simulink model "BendingMoments"  (R2026a)
settings: Solver=ode4  StartTime=0  StopTime=30  FixedStep=0.005  RelTol=1e-6
undefined symbols (not defined in the file or in its folder): mp
libraries: simulink x4, aerolibasang x3, aerolibadyn x1, aerolibatmos2 x1
settings Model: Creator=slugg  LastModifiedBy=slugg
settings DataIOCC: ReturnWorkspaceOutputsName=tp2dc5d62c_f7e5_43a9_8206_2db448d4c4c5

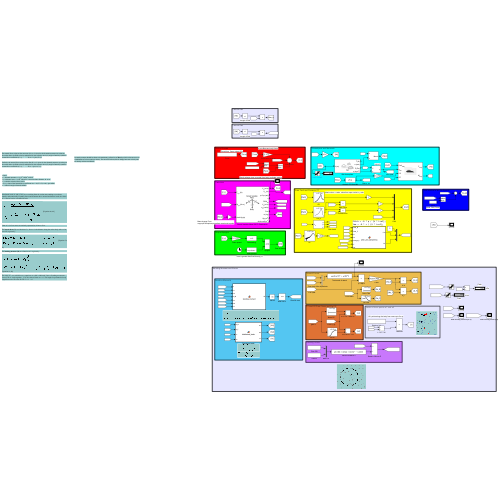
[thumbnail: Simulink's stored preview of the top-level diagram]
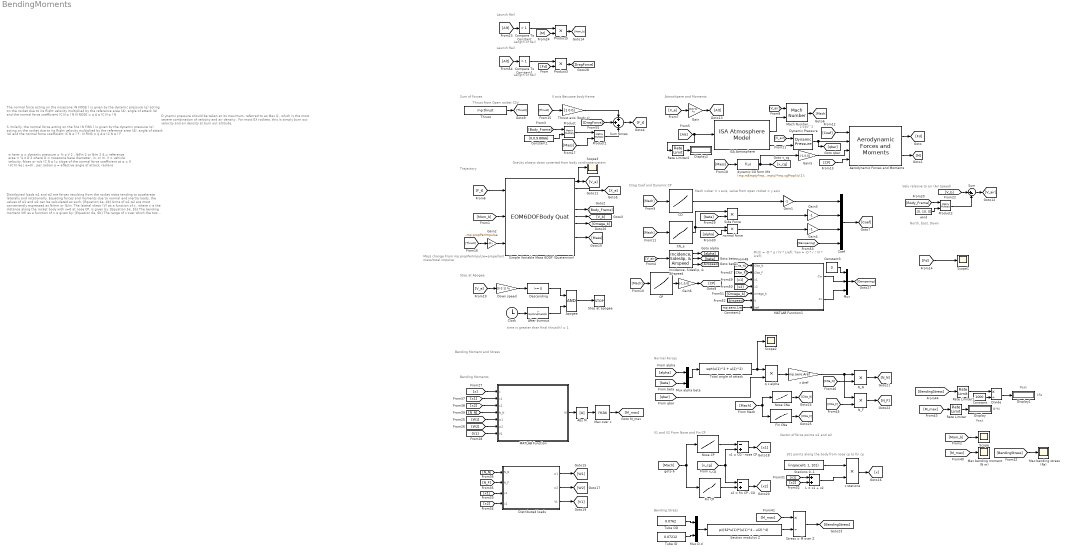
== system BendingMoments ==
  note: Bending Moment and Stress
  note: Pitch = -D * q / (V * Lref);
      | Yaw = -D * r / (V * Lref);
  note: Peak
  note: Peak
  note: N*M
  note: kPa
  note: Vector of force points w1 and w2
  note: 101 points along the body from nose cp to fin cp
  note: Normal Forces
  note: X1 and X2 From Nose and Fin CP
  note: Bending Moments
  note: Bending Stress
  note: Distributed loads w1 and w2 are forces resulting from the rocket mass tending to accelerate laterally and rotationally. Equating forces and moments due to normal and inertia loads, the values of w1 and w2 can be calculated as such:
      | [Equation 4a, 4b]
      | Units of w1,w2 are most conveniently expressed as N/mm or lb/in.
      | The lateral shear (V) as a function of x , where x is the distance along the rocket body with x=0 at nose CP, is given by:
      | [Equation 5a, 5b]
      | The bending moment (M) as a function of x is given by:
      | [Equation 6a, 6b]
      | The range of x over which the two equations are valid is indicated. Units of bending moment are N-mm or lb-in. In the equation , V1 is the value of shear at x=x1 . The length L represents the body length from nose CP to the fin CP: L = x1 + x2
  note: D ynamic pressure should be taken at its maximum, referred to as Max Q , which is the most severe combination of velocity and air density . For most EX rockets, this is simply burn out velocity and air density at burn out altitude.
  note: w here:
      | q = dynamic pressure = ½ ρ V 2 , lbf/in 2 or N/m 2
      | A = reference area = ¼ π D 2 where D = nosecone base diameter, in. or m.
      | V = vehicle velocity, ft/sec or m/s
      | (C N α )= slope of the normal force coefficient at α = 0 (∂C N /∂α | α=0) , per radian
      | α = effective angle of attack, radians
  note: S imilarly, the normal force acting on the fins (N FINS ) is given by the dynamic pressure (q) acting on the rocket due to its flight velocity multiplied by the reference area (A), angle of attack (α) and the normal force coefficient (C N α ) F : N FINS = q A α (C N α ) F
  note: The normal force acting on the nosecone (N NOSE ) is given by the dynamic pressure (q) acting on the rocket due to its flight velocity multiplied by the reference area (A), angle of attack (α) and the normal force coefficient (C N α ) N N NOSE = q A α (C N α ) N
  note: Mach nuber = x axis, value from open rocket = y axis
  note: time is greater than final thrust(t) = 1
  note: Mass change From
      | mp.propPerImpulse=propellant mass/total impulse
  note: X axis Becuase body frame
  note: Thrust from Open rocket CSV
  note: Gravity always down coverted from body cordinate system
  note: Length of Rail
  note: Launch Rail
  note: Velo relative to air (Air Speed)
  note: North, East, Down
  note: Atmoshpere and Moments
  note: Stop at Apogee
  note: Drag Coef and Dynamic CP
  note: Trajectory
  note: Sum of Forces
  note: 1/2pV^2
  note: Launch Rail
  note: Length of Rail
  Abs M : Abs  ZeroCross=off  SaturateOnIntegerOverflow=off
  "Aerodynamic Forces and Moments " : aerolibadyn/Aerodynamic Forces and Moments   inputAxes=Body  outputForceAxes=Body  outputMomentAxes=Body  S=mp.aero.Aref  b=mp.aero.Lref  cbar=mp.aero.Lref
  After burnout : simulink/Logic and Bit Operations/Compare To Constant  relop=>  const=mp.thrust(end,1)  OutDataTypeStr=boolean
  Apogee : Logic  AllPortsSameDT=off  OutDataTypeStr=boolean
  CD : Lookup_n-D  NumberOfTableDimensions=1  BreakpointsForDimension1=mp.aero.mach  Table=mp.aero.cd  ExtrapMethod=Clip  InternalRulePriority=Speed  RndMeth=Simplest
  CN_a : Lookup_n-D  NumberOfTableDimensions=1  BreakpointsForDimension1=[0.3, 0.4, 0.5, 0.6, 0.7, 0.8, 0.9, 1.0, 1.1, 1.2, 1.3, 1.4, 1.5, 1.6, 1.7]  Table=[9.822, 9.869, 9.931, 10.01, 10.108, 10.228, 10.374, 10.57, 10.867, 11.225, 11.509, 11.505, 10.944, 10.086, 9.424]  ExtrapMethod=Clip  InternalRulePriority=Speed  RndMeth=Simplest
  CP : Lookup_n-D  NumberOfTableDimensions=1  BreakpointsForDimension1=mp.aero.mach  Table=mp.aero.cp  ExtrapMethod=Clip  InternalRulePriority=Speed  RndMeth=Simplest
  Clock : Clock
  Coef : Mux  Inputs=[1,1,1,3]
  Compare To Constant : simulink/Logic and Bit Operations/Compare To Constant  relop=>  const=1  OutDataTypeStr=boolean
  Compare To Constant1 : simulink/Logic and Bit Operations/Compare To Constant  relop=>  const=1  OutDataTypeStr=boolean
  Constant : Constant  Value=1000
  Constant1 : Constant  Value=[0,0,9.8066]
  Constant2 : Constant  Value=mp.aero.Lref
  Constant3 : Constant  Value=0
  Descending : simulink/Logic and Bit Operations/Compare To Zero  relop=>=  OutDataTypeStr=boolean
  Display : Display
  Display1 : Display
  Display2 : Display
  Distributed loads : MATLAB Function  TreatAsAtomicUnit=on
  Divide : Product  Inputs=*/
  Down speed : Gain  Gain=[0 0 1]  Multiplication=Matrix(K*u)
  Dynamic Pressure : aerolibasang/Dynamic Pressure
  Fin CNa : Lookup_n-D  NumberOfTableDimensions=1  BreakpointsForDimension1=mp.coefs.mach  Table=mp.coefs.cnaFin  ExtrapMethod=Clip  InternalRulePriority=Speed  RndMeth=Simplest
  Fin CP : Lookup_n-D  NumberOfTableDimensions=1  BreakpointsForDimension1=mp.coefs.mach  Table=mp.coefs.cpFin  ExtrapMethod=Clip  InternalRulePriority=Speed  RndMeth=Simplest
  Gain : Gain  Gain=[0,0,-1]  Multiplication=Matrix(K*u)
  Gain1 : Gain  Gain=-1
  Gain2 : Gain  Gain=-mp.propPerImpulse
  Gain3 : Gain  Gain=-1
  Gain4 : Gain  Gain=-1
  Gain5 : Gain  Gain=[-1,0,0]
  Gain6 : Gain  Gain=[-1,0,0]
  ISA Atmosphere : aerolibatmos2/ISA Atmosphere Model  useExtended=off  action=None  custom=off  viscosityOut=off  g=9.80665  gamma=1.4  R=287.0531  L=0.0065  h_trop=11000  h_strat=20000  rho0=1.225  P0=101325  T0=288.15  h0=0  S=110.4  Tref=273.15  muref=1.716e-5
  "Incidence, Sideslip, & Airspeed" : aerolibasang/Incidence, Sideslip, & Airspeed
  L = x1 + x2 : Sum
  MATLAB Function : MATLAB Function  TreatAsAtomicUnit=on
  MATLAB Function1 : MATLAB Function  TreatAsAtomicUnit=on
  Mach Number : aerolibasang/Mach Number
  Max bending moment (N m) : Scope
      settings: ActiveDisplayYMinimum=0.0004903357093579766  ActiveDisplayYMaximum=4.5472668727370262
  Max bending stress (Pa) : Scope
      settings: MaximizeAxes=On  ActiveDisplayYMinimum=-17664.678991897163  ActiveDisplayYMaximum=566424.90728820558
  Max over x : MinMax  Function=max  ZeroCross=off
  Mux : Mux  Inputs=3
  Mux D d : Mux  Inputs=2
  Mux alpha beta : Mux  Inputs=2
  N_F : Product
  N_N : Product
  Nose CNa : Lookup_n-D  NumberOfTableDimensions=1  BreakpointsForDimension1=mp.coefs.mach  Table=mp.coefs.cnaNose  ExtrapMethod=Clip  InternalRulePriority=Speed  RndMeth=Simplest
  Nose CP : Lookup_n-D  NumberOfTableDimensions=1  BreakpointsForDimension1=mp.coefs.mach  Table=mp.coefs.cpNose  ExtrapMethod=Clip  InternalRulePriority=Speed  RndMeth=Simplest
  Product : Product  Multiplication=Matrix(*)
  Product1 : Product  Multiplication=Matrix(*)
  Product2 : Product  Multiplication=Matrix(*)
  Product3 : Product
  Product5 : Product
  Rate Limiter : RateLimiter  RisingSlewLimit=99999  FallingSlewLimit=0  SampleTimeMode=inherited
  Rate Limiter1 : RateLimiter  RisingSlewLimit=99999  FallingSlewLimit=0  SampleTimeMode=inherited
  Rate Limiter2 : RateLimiter  RisingSlewLimit=9999  FallingSlewLimit=0  SampleTimeMode=inherited
  Scope{,1..3} (4 alike) : Scope
      Scope settings: MaximizeAxes=On  ActiveDisplayYMinimum=-2.5627817572852805  ActiveDisplayYMaximum=2.573501952399988
      Scope1 settings: ActiveDisplayYMinimum=-439.08250593999844  ActiveDisplayYMaximum=776.726710241815
      Scope2 settings: ActiveDisplayYMinimum=-8.4391198295598269  ActiveDisplayYMaximum=9.3238404405735142  DataLoggingVariableName=ScopeData2
      Scope3 settings: ActiveDisplayYMinimum=-559.87555381280174  ActiveDisplayYMaximum=177.11836164042759  DataLoggingVariableName=ScopeData3
  Section modulus Z : Fcn  Expr=pi/(32*u(1))*(u(1)^4 - u(2)^4)
  Side Force : Product
  Simple Variable Mass 6DOF (Quaternion) : EOM6DOFBodyQuat  mtype=Simple Variable  eul_0=[0 deg2rad(87) 0]  mass_0=mp.mFull  mass_e=mp.mEmpty  mass_f=mp.mFull  inertia_e=mp.IEmpty  inertia_f=mp.IFull  mass_flag=on
  Stations 0..1 : Constant  Value=linspace(0, 1, 101)
  Stop at apogee : Stop
  Stress = M over Z : Product  Inputs=*/
  Sum : Sum  Inputs=|+-
  Sum forces : Sum  Inputs=+++
  Thrust : FromWorkspace  VariableName=mp.thrust  OutputAfterFinalValue=Setting to zero
  Thrust axis (body x) : Gain  Gain=[1 0 0]
  Total angle of attack : Fcn  Expr=sqrt(u(1)^2 + u(2)^2)
  Tube ID : Constant  Value=0.07212
  Tube OD : Constant  Value=0.0762
  dynamic CG form M/t : Fcn  Expr=(mp.mEmpty*mp.cgEmpty + (u(1) - mp.mEmpty)*mp.cgProp)/u(1);
  normal force : Product
  q x alpha : Product
  wind : Constant  Value=[0, 10, 0]
  x Aref : Gain  Gain=mp.aero.Aref
  x stations : Product
  x1 = CG - nose CP : Sum  Inputs=-+
  x2 = fin CP - CG : Sum  Inputs=-+
  wires:
  Thrust axis (body x)/1 -> Sum forces/1
  Gain5/1 -> "Aerodynamic Forces and Moments "/3
  [CP] -> "Aerodynamic Forces and Moments "/4
  ISA Atmosphere/4 -> Dynamic Pressure/2
  "Aerodynamic Forces and Moments "/2 -> [M]
  [Mom_b] -> Scope/1
  Dynamic Pressure/1 -> "Aerodynamic Forces and Moments "/2, [qbar]
  "Aerodynamic Forces and Moments "/1 -> [Fd]
  Simple Variable Mass 6DOF (Quaternion)/5 -> [Body_Frame]
  Product/1 -> Product1/1
  Constant1/1 -> Product/2
  [Body_Frame] -> Product/1
  [Mass] -> Product1/2
  [V_air] -> "Incidence, Sideslip, & Airspeed"/1
  [V_air] -> Mach Number/1
  ISA Atmosphere/2 -> Mach Number/2
  CD/1 -> Gain1/1
  Sum forces/1 -> [F_t]
  [F_t] -> Simple Variable Mass 6DOF (Quaternion)/1
  Simple Variable Mass 6DOF (Quaternion)/6 -> [V_b]
  Simple Variable Mass 6DOF (Quaternion)/2 -> [X_e]
  [X_e] -> Gain/1
  [V_air] -> Dynamic Pressure/1
  Mach Number/1 -> [Mach]
  [Mach] -> CD/1
  [Mach] -> CP/1
  [Mach] -> CN_a/1
  CN_a/1 -> normal force/1, Side Force/1
  Side Force/1 -> Gain3/1
  normal force/1 -> Gain4/1
  [Dampening] -> Coef/4
  Gain3/1 -> Coef/2
  Gain4/1 -> Coef/3
  Gain1/1 -> Coef/1
  CP/1 -> Gain6/1
  [Fd] -> Scope1/1
  "Incidence, Sideslip, & Airspeed"/2 -> [beta]
  "Incidence, Sideslip, & Airspeed"/1 -> [alpha]
  Thrust/1 -> [Thrust]
  [Thrust] -> Thrust axis (body x)/1
  [Thrust] -> Gain2/1
  [Mass] -> dynamic CG form M/t/1
  dynamic CG form M/t/1 -> Gain5/1, [x_cg]
  Gain6/1 -> [CP]
  Down speed/1 -> Descending/1
  Clock/1 -> After burnout/1
  Descending/1 -> Apogee/1
  After burnout/1 -> Apogee/2
  Apogee/1 -> Stop at apogee/1
  Simple Variable Mass 6DOF (Quaternion)/1 -> Scope3/1, [V_e]
  [V_e] -> Down speed/1
  wind/1 -> Product2/2
  [Body_Frame] -> Product2/1
  Product2/1 -> Sum/2
  [V_b] -> Sum/1
  Sum/1 -> [V_air]
  Gain/1 -> [Alt]
  [Alt] -> Rate Limiter2/1, ISA Atmosphere/1
  [Alt] -> Compare To Constant/1
  Compare To Constant/1 -> Product5/1
  [M] -> Product5/2
  Product5/1 -> [Mom_b]
  [alpha] -> Mux alpha beta/1
  [beta] -> Mux alpha beta/2
  Mux alpha beta/1 -> Total angle of attack/1
  Total angle of attack/1 -> Scope2/1, q x alpha/1
  q x alpha/1 -> x Aref/1
  [Mach] -> Nose CNa/1, Fin CNa/1
  [Mach] -> Nose CP/1, Fin CP/1
  Nose CP/1 -> x1 = CG - nose CP/1
  [x_cg] -> x1 = CG - nose CP/2, x2 = fin CP - CG/1
  Fin CP/1 -> x2 = fin CP - CG/2
  Stations 0..1/1 -> x stations/1
  L = x1 + x2/1 -> x stations/2
  MATLAB Function/1(M) -> Abs M/1
  Tube OD/1 -> Mux D d/1
  Tube ID/1 -> Mux D d/2
  Mux D d/1 -> Section modulus Z/1
  Section modulus Z/1 -> Stress = M over Z/2
  [qbar] -> q x alpha/2
  Distributed loads/1(w1) -> [W1]
  [W1] -> MATLAB Function/5(w1)
  [W2] -> MATLAB Function/6(w2)
  Distributed loads/3(V1) -> [V1]
  Distributed loads/2(w2) -> [W2]
  [V1] -> MATLAB Function/7(V1)
  x stations/1 -> [x]
  [x] -> MATLAB Function/1(x)
  [beta] -> Side Force/2
  [alpha] -> normal force/2
  Coef/1 -> [Coef]
  x1 = CG - nose CP/1 -> [x1]
  [x1] -> L = x1 + x2/1
  x2 = fin CP - CG/1 -> [x2]
  [x2] -> L = x1 + x2/2
  [x1] -> Distributed loads/3(x1)
  [x2] -> Distributed loads/4(x2)
  N_N/1 -> [N_N]
  N_F/1 -> [N_F]
  [N_N] -> Distributed loads/1(N_N)
  [N_F] -> Distributed loads/2(N_F)
  [x1] -> MATLAB Function/2(x1)
  [x2] -> MATLAB Function/3(x2)
  [N_N] -> MATLAB Function/4(N_N)
  [M_max] -> Max bending moment (N m)/1
  [M_max] -> Stress = M over Z/1
  Stress = M over Z/1 -> [BendingStress]
  [BendingStress] -> Max bending stress (Pa)/1
  x Aref/1 -> N_F/1, N_N/1
  [M_max] -> Rate Limiter/1
  Rate Limiter/1 -> Display/1
  [BendingStress] -> Rate Limiter1/1
  Constant/1 -> Divide/2
  Rate Limiter1/1 -> Divide/1
  Divide/1 -> Display1/1
  Rate Limiter2/1 -> Display2/1
  Fin CNa/1 -> [CNa_F]
  Nose CNa/1 -> [CNa_N]
  [CNa_N] -> N_N/2
  [CNa_F] -> N_F/2
  [CNa_N] -> MATLAB Function1/1(CNa_N)
  [CNa_F] -> MATLAB Function1/2(CNa_F)
  [x1] -> MATLAB Function1/3(x1)
  [x2] -> MATLAB Function1/4(x2)
  [Omega_b] -> MATLAB Function1/5(omega_b)
  "Incidence, Sideslip, & Airspeed"/3 -> [Airspeed]
  [Airspeed] -> MATLAB Function1/6(V)
  Constant2/1 -> MATLAB Function1/7(lref)
  MATLAB Function1/1(Cm) -> Mux/2
  MATLAB Function1/2(Cn) -> Mux/3
  Constant3/1 -> Mux/1
  Mux/1 -> [Dampening]
  Abs M/1 -> Max over x/1
  Max over x/1 -> [M_max]
  [Coef] -> "Aerodynamic Forces and Moments "/1
  Simple Variable Mass 6DOF (Quaternion)/7 -> [Omega_b]
  Simple Variable Mass 6DOF (Quaternion)/9 -> [Mass]
  [Mom_b] -> Simple Variable Mass 6DOF (Quaternion)/2
  Gain2/1 -> Simple Variable Mass 6DOF (Quaternion)/3
  Compare To Constant1/1 -> Product3/1
  Product3/1 -> [DragForce]
  [Alt] -> Compare To Constant1/1
  [Fd] -> Product3/2
  [DragForce] -> Sum forces/2
  ? -> ?
  ? -> ?
  Product1/1 -> Sum forces/3

== matlab function BendingMoments/Distributed loads ==
  data: N_N input; w1 output; N_F input; x1 input; x2 input; w2 output; V1 output
function [w1, w2, V1] = distributed_loads(N_N, N_F, x1, x2)

w2 = (N_F*(2*x2 + x1) - N_N*x1) / (x2^2 + x1*x2);
w1 = (N_N + N_F - w2*x2) / x1;
V1 = N_N - w1*x1;
end

== matlab function BendingMoments/MATLAB Function ==
  data: x input; M output; x1 input; x2 input; N_N input; w1 input; w2 input; V1 input
function M = bending_moment(x, x1, x2, N_N, w1, w2, V1)

L = x1 + x2;
M = zeros(size(x));

i1 = (x >= 0) & (x <= x1);
M(i1) = N_N .* x(i1) - w1 .* x(i1).^2 ./ 2;

i2 = (x > x1) & (x <= L);
M(i2) = V1 .* x(i2) ...
      + w2 .* (x1 .* x(i2) + 0.5 .* L.^2 - 0.5 .* x(i2).^2) ...
      - L .* (V1 + w2 .* x1);
end

== matlab function BendingMoments/MATLAB Function1 ==
  data: CNa_N input; Cm output; CNa_F input; x1 input; x2 input; omega_b input; V input; lref input; Cn output
function [Cm, Cn] = pitch_yaw_dampening(CNa_N, CNa_F, x1, x2, omega_b, V, lref)

V = max(V, 1);
D = CNa_N * x1^2 + CNa_F * x2^2;

q = omega_b(2);
r = omega_b(3);

Cm = -D * q / (V * lref);
Cn = -D * r / (V * lref);
end
